simulink model "circuito_TP1_TL081"  (R2025b)
settings: Solver=ode23t  StartTime=0.0  StopTime=0.1  MaxStep=1e-5  RelTol=1e-6
InitFcn:
  | % Valores de la Fig. 1, solo si no estan definidos en el workspace
  | if ~exist('R1','var'), R1 = 100e3; end
  | if ~exist('R2','var'), R2 = 47e3; end
  | if ~exist('R3','var'), R3 = 1e3; end
  | if ~exist('R4','var'), R4 = 1e3; end
  | if ~exist('R5','var'), R5 = 1e3; end
  | if ~exist('R6','var'), R6 = 1e3; end
  | if ~exist('R7','var'), R7 = 10e3; end
  | if ~exist('R8','var'), R8 = 1e3; end
  | if ~exist('R9','var'), R9 = 1e3; end
  | if ~exist('C1','var'), C1 = 0.1e-6; end
  | if ~exist('C2','var'), C2 = 0.1e-6; end
  | if ~exist('Vin','var'), Vin = 1; end
undefined symbols (not defined in the file): R1, R2, R3, R4, R5, R6, R7, R8, R9, Vin
libraries: fl_lib x21, nesl_utility x4, ee_lib x3
settings Model: Creator=ruben  LastModifiedBy=ruben

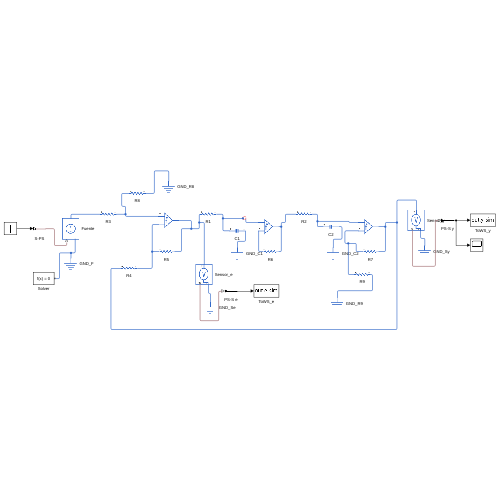
[thumbnail: Simulink's stored preview of the top-level diagram]
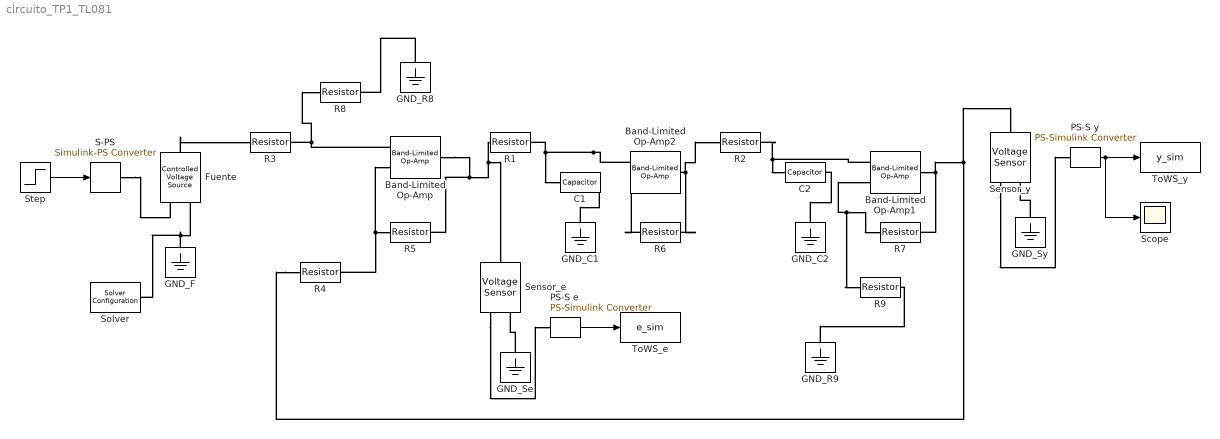
== system circuito_TP1_TL081 ==
  Band-Limited Op-Amp : ee_lib/Integrated Circuits/Band-Limited Op-Amp  A=2e5  Rin=1e12 Ohm  Rout=0 Ohm  Vmin=-8.5 V  Vmax=8.5 V  Vdotmax=13e6 V/s  f=15 Hz  V0=0 V
  Band-Limited Op-Amp1 : ee_lib/Integrated Circuits/Band-Limited Op-Amp  A=2e5  Rin=1e12 Ohm  Rout=0 Ohm  Vmin=-8.5 V  Vmax=8.5 V  Vdotmax=13e6 V/s  f=15 Hz  V0=0 V
  Band-Limited Op-Amp2 : ee_lib/Integrated Circuits/Band-Limited Op-Amp  A=2e5  Rin=1e12 Ohm  Rout=0 Ohm  Vmin=-8.5 V  Vmax=8.5 V  Vdotmax=13e6 V/s  f=15 Hz  V0=0 V
  C1 : fl_lib/Electrical/Electrical Elements/Capacitor  c=C1 F  r=1e-6 Ohm  g=0 1/Ohm  i_specify=off  i_priority=None  i=0 A  i_nominal_specify=off  i_nominal_value=1  i_nominal_unit=A  v_specify=off  v_priority=None  v=0 V  v_nominal_specify=off  v_nominal_value=1  v_nominal_unit=V  vc_specify=on  vc_priority=High  vc=0 V  vc_nominal_specify=off  vc_nominal_value=1  vc_nominal_unit=V
  C2 : fl_lib/Electrical/Electrical Elements/Capacitor  c=C2 F  r=1e-6 Ohm  g=0 1/Ohm  i_specify=off  i_priority=None  i=0 A  i_nominal_specify=off  i_nominal_value=1  i_nominal_unit=A  v_specify=off  v_priority=None  v=0 V  v_nominal_specify=off  v_nominal_value=1  v_nominal_unit=V  vc_specify=on  vc_priority=High  vc=0 V  vc_nominal_specify=off  vc_nominal_value=1  vc_nominal_unit=V
  Fuente : fl_lib/Electrical/Electrical Sources/Controlled Voltage Source
  GND_C1 : fl_lib/Electrical/Electrical Elements/Electrical Reference
  GND_C2 : fl_lib/Electrical/Electrical Elements/Electrical Reference
  GND_F : fl_lib/Electrical/Electrical Elements/Electrical Reference
  GND_R8 : fl_lib/Electrical/Electrical Elements/Electrical Reference
  GND_R9 : fl_lib/Electrical/Electrical Elements/Electrical Reference
  GND_Se : fl_lib/Electrical/Electrical Elements/Electrical Reference
  GND_Sy : fl_lib/Electrical/Electrical Elements/Electrical Reference
  PS-S e : nesl_utility/PS-Simulink Converter  PhysicalDomain=network_engine_domain  SubClassName=ps_output  LeftPortType=input  RightPortType=output  PseudoPeriodic=off  Frequencies=[]  VectorFormat=inherit  Unit=inherit  AffineConversion=off
  PS-S y : nesl_utility/PS-Simulink Converter  PhysicalDomain=network_engine_domain  SubClassName=ps_output  LeftPortType=input  RightPortType=output  PseudoPeriodic=off  Frequencies=[]  VectorFormat=inherit  Unit=inherit  AffineConversion=off
  R1 : fl_lib/Electrical/Electrical Elements/Resistor  R=R1 Ohm  i_specify=off  i_priority=None  i=0 A  i_nominal_specify=off  i_nominal_value=1  i_nominal_unit=A  v_specify=off  v_priority=None  v=0 V  v_nominal_specify=off  v_nominal_value=1  v_nominal_unit=V
  R2 : fl_lib/Electrical/Electrical Elements/Resistor  R=R2 Ohm  i_specify=off  i_priority=None  i=0 A  i_nominal_specify=off  i_nominal_value=1  i_nominal_unit=A  v_specify=off  v_priority=None  v=0 V  v_nominal_specify=off  v_nominal_value=1  v_nominal_unit=V
  R3 : fl_lib/Electrical/Electrical Elements/Resistor  R=R3 Ohm  i_specify=off  i_priority=None  i=0 A  i_nominal_specify=off  i_nominal_value=1  i_nominal_unit=A  v_specify=off  v_priority=None  v=0 V  v_nominal_specify=off  v_nominal_value=1  v_nominal_unit=V
  R4 : fl_lib/Electrical/Electrical Elements/Resistor  R=R4 Ohm  i_specify=off  i_priority=None  i=0 A  i_nominal_specify=off  i_nominal_value=1  i_nominal_unit=A  v_specify=off  v_priority=None  v=0 V  v_nominal_specify=off  v_nominal_value=1  v_nominal_unit=V
  R5 : fl_lib/Electrical/Electrical Elements/Resistor  R=R5 Ohm  i_specify=off  i_priority=None  i=0 A  i_nominal_specify=off  i_nominal_value=1  i_nominal_unit=A  v_specify=off  v_priority=None  v=0 V  v_nominal_specify=off  v_nominal_value=1  v_nominal_unit=V
  R6 : fl_lib/Electrical/Electrical Elements/Resistor  R=R6 Ohm  i_specify=off  i_priority=None  i=0 A  i_nominal_specify=off  i_nominal_value=1  i_nominal_unit=A  v_specify=off  v_priority=None  v=0 V  v_nominal_specify=off  v_nominal_value=1  v_nominal_unit=V
  R7 : fl_lib/Electrical/Electrical Elements/Resistor  R=R7 Ohm  i_specify=off  i_priority=None  i=0 A  i_nominal_specify=off  i_nominal_value=1  i_nominal_unit=A  v_specify=off  v_priority=None  v=0 V  v_nominal_specify=off  v_nominal_value=1  v_nominal_unit=V
  R8 : fl_lib/Electrical/Electrical Elements/Resistor  R=R8 Ohm  i_specify=off  i_priority=None  i=0 A  i_nominal_specify=off  i_nominal_value=1  i_nominal_unit=A  v_specify=off  v_priority=None  v=0 V  v_nominal_specify=off  v_nominal_value=1  v_nominal_unit=V
  R9 : fl_lib/Electrical/Electrical Elements/Resistor  R=R9 Ohm  i_specify=off  i_priority=None  i=0 A  i_nominal_specify=off  i_nominal_value=1  i_nominal_unit=A  v_specify=off  v_priority=None  v=0 V  v_nominal_specify=off  v_nominal_value=1  v_nominal_unit=V
  S-PS : nesl_utility/Simulink-PS Converter  PhysicalDomain=network_engine_domain  SubClassName=ps_input  LeftPortType=input  RightPortType=output  PseudoPeriodic=off  Frequencies=[]  NoiseDistribution=none  NoiseParameters=[]  Unit=1  AffineConversion=off  FilteringAndDerivatives=provide  SimscapeFilterOrder=1  InputFilterTimeConstant=0.001  UdotUserProvided=0
  Scope : Scope
      settings: ActiveDisplayYMinimum=-1  ActiveDisplayYMaximum=1
  Sensor_e : fl_lib/Electrical/Electrical Sensors/Voltage Sensor
  Sensor_y : fl_lib/Electrical/Electrical Sensors/Voltage Sensor
  Solver : nesl_utility/Solver Configuration  PhysicalDomain=network_engine_domain  SubClassName=solver  LeftPortType=input  RightPortType=generic  Tones=[]  Harmonics=[]  SimulateNoise=off  Profile=off  UseLocalSampling=off  EnableSwitchedLinearOptims=on  FrequencyDomain=off  UseCCode=off  RelTol=0.001  AbsTol=0.001  MinStep=1e-09  ToWorkspace=off  RevertToSquareIcSolve=off  NumHomotopyIterations=100  PhasorMode=off  PhasorModeNumHarmonics=1  ConsistencySolver=NEWTON_XTOL_AFTER_FTOL  IndexReductionMethod=DerivativeReplacement  DoDC=off  ResidualTolerance=1e-09  ConsistencyTolSource=GLOBAL  ConsistencyAbsTol=0.001  ConsistencyRelTol=0.001  ConsistencyTolFactor=0.001  UseLocalSolver=off  LocalSolverChoice=NE_BACKWARD_EULER_ADVANCER  ResolveIndetEquations=on  FunctionEvalNumThread=1  LocalSolverSampleTime=0.001  DoFixedCost=off  MaxNonlinIter=3  MaxModeIter=2  ComputeImpulses=off  ImpulseIterations=2  LinearAlgebra=auto  LinearAlgebraNumThread=0  EquationFormulation=NE_TIME_EF  DelaysMemoryBudget=1024  AutomaticFiltering=on  FilteringTimeConstant=0.001  PartitionStorageMethod=AS_NEEDED  PartitionMemoryBudget=1024  PartitionMethod=ROBUST  MultibodyUseLocalSolver=off  MultibodyLocalSolverChoice=ODE1  MultibodyLocalSolverSampleTime=0.001
  Step : Step  Time=0  After=Vin  SampleTime=0
  ToWS_e : ToWorkspace  VariableName=e_sim  SaveFormat=Timeseries  SampleTime=-1
  ToWS_y : ToWorkspace  VariableName=y_sim  SaveFormat=Timeseries  SampleTime=-1
  wires:
  Step/1 -> S-PS/1
  PS-S y/1 -> ToWS_y/1, Scope/1
  PS-S e/1 -> ToWS_e/1
  connections:
  Fuente/LConn1 -- R3/LConn1
  R3/RConn1 -- Band-Limited Op-Amp/LConn1 -- R8/LConn1
  R5/RConn1 -- Band-Limited Op-Amp/RConn1 -- Sensor_e/LConn1 -- R1/LConn1
  C1/LConn1 -- Band-Limited Op-Amp2/LConn1 -- R1/RConn1
  R6/LConn1 -- Band-Limited Op-Amp2/LConn2
  R6/RConn1 -- R2/LConn1 -- Band-Limited Op-Amp2/RConn1
  R2/RConn1 -- C2/LConn1 -- Band-Limited Op-Amp1/LConn1
  R9/LConn1 -- Band-Limited Op-Amp1/LConn2 -- R7/LConn1
  R4/LConn1 -- R7/RConn1 -- Band-Limited Op-Amp1/RConn1 -- Sensor_y/LConn1
  GND_F/LConn1 -- Fuente/RConn2 -- Solver/RConn1
  GND_R8/LConn1 -- R8/RConn1
  GND_C1/LConn1 -- C1/RConn1
  GND_C2/LConn1 -- C2/RConn1
  GND_R9/LConn1 -- R9/RConn1
  GND_Sy/LConn1 -- Sensor_y/RConn2
  GND_Se/LConn1 -- Sensor_e/RConn2
  S-PS/RConn1 -- Fuente/RConn1
  Sensor_y/RConn1 -- PS-S y/LConn1
  Sensor_e/RConn1 -- PS-S e/LConn1
  R4/RConn1 -- Band-Limited Op-Amp/LConn2 -- R5/LConn1
